simulink model "emso"  (Simulink 7.1)
settings: Solver=ode45  StartTime=0.0  StopTime=5  RelTol=1e-3
settings Model: Creator=lades  LastModifiedBy=W7
settings DataIOCC: ExternalInput=Az
settings DebuggingCC: SaveWithDisabledLinksMsg=none  SaveWithParameterizedLinksMsg=none  CheckSSInitialOutputMsg=off  SolverPrmCheckMsg=none  MultiTaskCondExecSysMsg=none  Int32ToFloatConvMsg=none  ModelReferenceDataLoggingMessage=none

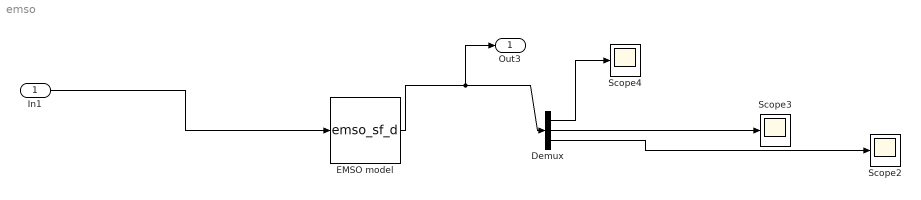
== system emso ==
  In1 : Inport  OutDataType=sfix(16)  OutScaling=2^0
  Demux : Demux  Outputs=3
  EMSO model : S-Function  FunctionName=emso_sf_d  Parameters='Problem_2F.ems',5,3,0.5  EnableBusSupport=off
  Scope2 : Scope
      settings: TimeRange=5  YMin=0  YMax=45
  Scope3 : Scope
      settings: TimeRange=5  YMin=0  YMax=45  SaveName=ScopeData2
  Scope4 : Scope
      settings: TimeRange=5  YMin=0  YMax=45  SaveName=ScopeData3
  Out3 : Outport
  wires:
  EMSO model/1 -> Demux/1, Out3/1
  Demux/3 -> Scope2/1
  Demux/2 -> Scope3/1
  Demux/1 -> Scope4/1
  In1/1 -> EMSO model/1
